simulink model "bicopter_startAngelo"  (R2026b)
settings: Solver=VariableStepAuto  StopTime=50
PreLoadFcn:
  | addpath("Support_Files/")
  | modelParams
model workspace (MAT data in the model file):
  TwinPivotDamping = 5.5e-05
  TwinThrustCoefficient = 0.9085
undefined symbols (not defined in the file or in its folder): battVoltage, MassVals, smiData, X, Y, Z
libraries: sm_lib x20, fl_lib x11, nesl_utility x4, sdl_lib x2, ee_lib x2, slpidlib x1, cstblocks_lti x1
(part 1 of 2)
settings Model: Creator=aredfear  LastModifiedBy=ayeo
settings RTWCC: GPUComputeCapability=5.0
settings SimscapeCC: SimscapeUseEnergyAccounting=off
settings ExplorerConfigSet: InternalSimMechanicsExplorerSettings=|
  | <ExplorerConfiguration>
  | 
  |   <canonicalview>default</canonicalview>
  | 
  |   <TilePanel>
  |     <TileInfo>
  |       <Tiles Columns="1" Count="1" Height="310" Rows="1" Width="757">
  |         <Row Weight="1"/>
  |         <Column Weight="1"/>
  |         <Tile Height="1" Width="1" X="0" Y="0"/>
  |       </Tiles>
  |     </TileInfo>
  |     <SceneInfo>
  |       <SceneViewer>
  |         <IsThisViewStd>
  |           <IsStandardView>off</IsStandardView>
  |           <StandardViewName>Front</StandardViewName>
  |         </IsThisViewStd>
  |         <BGColor>
  |           <R>1</R>
  |           <G>1</G>
  |           <B>1</B>
  |           <A>1</A>
  |         </BGColor>
  |         <Camera>
  |           <DoPerspective>off</DoPerspective>
  |           <Position>
  |             <X>0.27879065959295879</X>
  |             <Y>-2.0709674160574254</Y>
  |             <Z>0.54548044125818385</Z>
  |           </Position>
  |           <Center>
  |             <X>-0.0098286292275114144</X>
  |             <Y>0.00045902017735405254</Y>
  |             <Z>0.055789039094021275</Z>
  |           </Center>
  |           <Up>
  |             <X>-0.012086790678740725</X>
  |             <Y>0.22844965094818886</Y>
  |             <Z>0.97348069650750602</Z>
  |           </Up>
  |           <XLim>0.10544914134742404</XLim>
  |           <YLim>0.10544914134742404</YLim>
  |           <ViewLimDist>0.01</ViewLimDist>
  |         </Camera>
  |       </SceneViewer>
  |     </SceneInfo>
  |   </TilePanel>
  | 
  |   <MechEditorPanel>
  |     <GfxPanelCameraMap/>
  |     <Cameras/>
  |     <VideoCreator>
  |       <IncludeTiles>All</IncludeTiles>
  |       <IncludeTime>on</IncludeTime>
  |       <IncludeWorldFrame>off</IncludeWorldFrame>
  |       <PlaybackSpeedRatio>1</PlaybackSpeedRatio>
  |       <FrameRate>30</FrameRate>
  |       <FrameSize>auto</FrameSize>
  |       <VideoFormat>UncompressedAVI</VideoFormat>
  |     </VideoCreator>
  |   </MechEditorPanel>
  | 
  |   <PlaybackSettings>
  |     <PlaybackSpeedFactor>1</PlaybackSpeedFactor>
  |   </PlaybackSettings>
  | 
  | </ExplorerConfiguration>

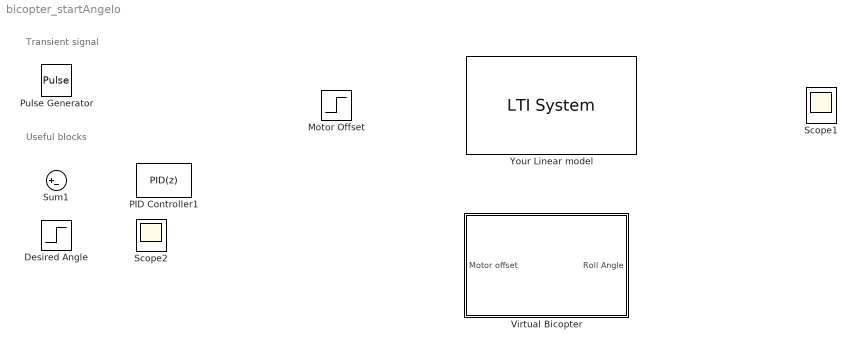
== system bicopter_startAngelo ==
  note: Useful blocks
  note: Transient signal
  Desired Angle : Step  FinalValue=20 * pi / 180  SampleTime=0
  Motor Offset : Step  FinalValue=5  SampleTime=0
  PID Controller1 : slpidlib/PID Controller  Controller=PID  Form=Parallel  TimeDomain=Discrete-time  UseExternalTs=off  SampleTime=0.001  IntegratorMethod=Forward Euler  FilterMethod=Forward Euler  ControllerParametersSource=internal  P=1  I=1  UseKiTs=off  D=0  UseExternalDerivativeSource=off  N=100  UseFilter=on  TunerSelectOption=Transfer Function Based (PID Tuner App)  InitialConditionSource=internal  InitialConditionForIntegrator=0  InitialConditionForFilter=0  DifferentiatorICPrevScaledInput=0  ExternalReset=none  TrackingMode=off  Kt=1  LimitOutput=on  SatLimitsSource=internal  UpperSaturationLimit=30  LowerSaturationLimit=-30  LinearizeAsGain=on  AntiWindupMode=clamping  Kb=1  LimitIntegrator=off  UpperIntegratorSaturationLimit=inf  LowerIntegratorSaturationLimit=-inf  POutMin=[]  POutMax=[]  IOutMin=[]  IOutMax=[]  DOutMin=[]  DOutMax=[]  NOutMin=[]  NOutMax=[]  SumOutMin=[]  SumOutMax=[]  SaturationOutMin=[]  SaturationOutMax=[]  PParamMin=[]  PParamMax=[]  IParamMin=[]  IParamMax=[]  DParamMin=[]  DParamMax=[]  NParamMin=[]  NParamMax=[]  KbParamMin=[]  KbParamMax=[]  KtParamMin=[]  KtParamMax=[]  KbOutMin=[]  KbOutMax=[]  KtOutMin=[]  KtOutMax=[]  IntegratorOutMin=[]  IntegratorOutMax=[]  FilterOutMin=[]  FilterOutMax=[]  SumI1OutMin=[]  SumI1OutMax=[]  SumI2OutMin=[]  SumI2OutMax=[]  SumI3OutMin=[]  SumI3OutMax=[]  SumI4OutMin=[]  SumI4OutMax=[]  SumDOutMin=[]  SumDOutMax=[]  DifferentiatorOutMin=[]  DifferentiatorOutMax=[]  FilterDiffOutCoefMin=[]  FilterDiffOutCoefMax=[]  ReciprocalOutMin=[]  ReciprocalOutMax=[]  SumDenOutMin=[]  SumDenOutMax=[]  SumNumOutMin=[]  SumNumOutMax=[]  DivideOutMin=[]  DivideOutMax=[]  UdiffTsProdOutMin=[]  UdiffTsProdOutMax=[]  NTsProdOutMin=[]  NTsProdOutMax=[]  UintegralTsProdOutMin=[]  UintegralTsProdOutMax=[]  UngainTsProdOutMin=[]  UngainTsProdOutMax=[]  ClampingZeroOutDataTypeStr=Inherit: Inherit via back propagation  ClampingZeroOutMin=[]  ClampingZeroOutMax=[]  FilterDenConstantOutDataTypeStr=Inherit: Inherit via back propagation  FilterDenConstantOutMin=[]  FilterDenConstantOutMax=[]  PCopyOutDataTypeStr=Inherit: Inherit via back propagation  PCopyOutMin=[]  PCopyOutMax=[]  NCopyOutDataTypeStr=Inherit: Inherit via back propagation  NCopyOutMin=[]  NCopyOutMax=[]  IntegratorContinuousStateAttributes=''  IntegratorStateMustResolveToSignalObject=off  IntegratorRTWStateStorageClass=Auto  FilterContinuousStateAttributes=''  FilterStateMustResolveToSignalObject=off  FilterRTWStateStorageClass=Auto  ParallelPVariant=InternalParameters  IdealPVariant=Disabled  IVariant=InternalParameters  DVariant=InternalParameters  IntegratorVariant=Discrete  SatVariant=Enabled  AWVariant=DiscClampingParallel  PCopyVariant=Disabled  TRVariant=Disabled  FdbkBlocksVariant=Forward  IdealPFdbkVariant=Disabled  SatFdbkVariant=Disabled  DerivativeFilterVariant=ForwardEulerFilter  NVariant=InternalParameters  NCopyVariant=Disabled  FilterICVariant=InternalICsFilter  IntegratorICVariant=InternalICs  ExternalResetVariant=Disabled  TRSumVariant=Passthrough  SumFdbkVariant=Disabled  SumVariant=Sum_PID  TsampFilterVariant=InternalTs  TsampNgainVariant=Passthrough  TsampIntegralVariant=Disabled_SignalSpec  ExternalSaturationOutDataTypeStr=Inherit: Same as second input  DerivativeSourceVariant=ErrorSignal  PreIntVariant=InternalPreInt
  Pulse Generator : DiscretePulseGenerator  PulseType=Time based  Amplitude=20 * pi / 180  Period=50  PulseWidth=50  PhaseDelay=10
  Scope1 : Scope
      settings: ActiveDisplayYMinimum=-0.043692144868254922  ActiveDisplayYMaximum=0.39270562765076822
  Scope2 : Scope
      settings: DataLoggingVariableName=ScopeData2
  Sum1 : Sum  Inputs=|+-
  Virtual Bicopter : Subsystem
      mask Display: image('bicopter.png');
  Your Linear model : cstblocks_lti/LTI System  sys=myModel  IC=[]  PadeOrder=0

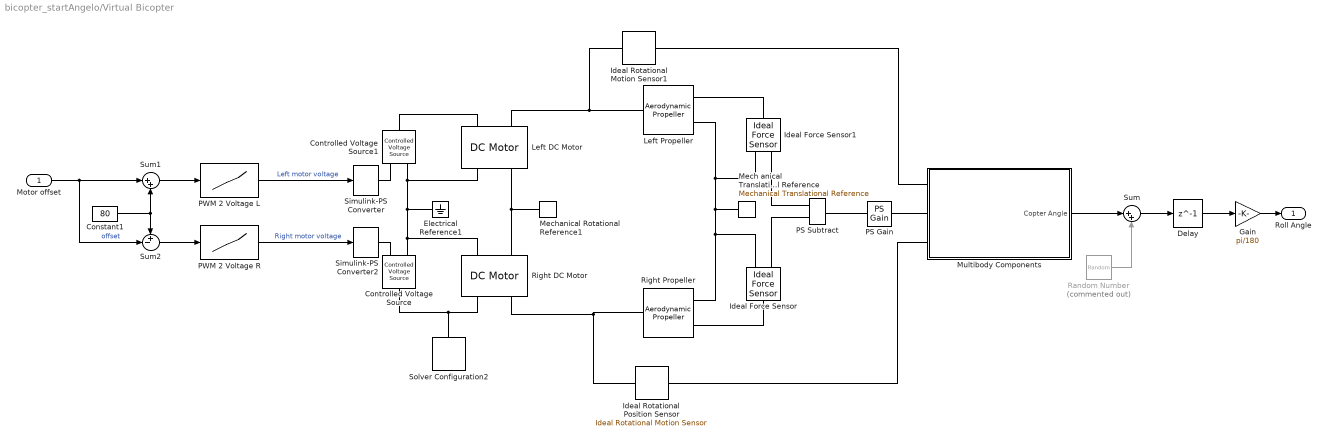
== system bicopter_startAngelo/Virtual Bicopter ==
  Motor offset : Inport
  Constant1 : Constant  Value=80
  Controlled Voltage Source : fl_lib/Electrical/Electrical Sources/Controlled Voltage Source
  Controlled Voltage Source1 : fl_lib/Electrical/Electrical Sources/Controlled Voltage Source
  Delay : Delay  DelayLength=1
  Electrical Reference1 : fl_lib/Electrical/Electrical Elements/Electrical Reference
  Gain : Gain  Gain=pi/180
  Ideal Force Sensor : fl_lib/Mechanical/Mechanical Sensors/Ideal Force Sensor
  Ideal Force Sensor1 : fl_lib/Mechanical/Mechanical Sensors/Ideal Force Sensor
  Ideal Rotational Motion Sensor1 : fl_lib/Mechanical/Mechanical Sensors/Ideal Rotational Motion Sensor  reference=foundation.enum.MeasurementReference.absolute  acceleration_port=false  velocity_port=false  position_port=true  wrap_angle=simscape.enum.onoff.off  offset=0 rad
  Ideal Rotational Position Sensor : fl_lib/Mechanical/Mechanical Sensors/Ideal Rotational Motion Sensor  reference=foundation.enum.MeasurementReference.absolute  acceleration_port=false  velocity_port=false  position_port=true  wrap_angle=false  offset=0 rad
  Left Propeller : sdl_lib/Engines & Motors/Aerodynamic Propeller  parameterization=sdl.enum.AerodynamicPropellerParameterization.Constant  enable_collective_pitch_control=false  enable_transverse_flow=false  direction=sdl.enum.PropellerDirection.Positive  root_pitch=0 deg  D=.02 m  kt_const=TwinThrustCoefficient  kp_const=0.13  kt_poly_fixed=[.002, .0006, -.0509, .0617]  kp_poly_fixed=[-.0752, .0577, -.0622, .16]  pitch_angle_TLU=[-15, 15, 25, 35, 45] deg  kt_poly_TLU=[.0002, -.00041, -.036, .03; .00026, -.00056, -.048, .04; .002, .00063, -.051, .062; .0014, -.0016, -.048, .087; .00087, -.0036, -.041, .12]  kp_poly_TLU=[-.1, .031, .0055, .088; -.081, -.025, .0044, .07; -.075, .058, -.062, .16; -.052, .065, -.08, .3; -.031, .057, -.069, .4]  J_TLU=[.01, .3, .625, 1.55, 2, 2.6]  kt_TLU_1D=[.0614, .0473, .0318, -.0127, -.0343, -.063]  kp_TLU_1D=[.1496, .1314, .116, -.0521, -.1503, -.2813]  kt_TLU_2D=[.00019, .013, .0048, -.017, -.03, -.045; .00039, .025, .0096, -.037, -.06, -.09; .00061, .047, .032, -.013, -.034, -.063; .00086, .072, .057, .014, -.0076, -.036; .12, .104, .09, .049, .029, .0019]  kp_TLU_2D=[.029, .029, .016, .06, .009, -.16; .059, .054, .031, -.12, -.19, -.29; .15, .13, .12, -.052, -.15, -.28; .26, .24, .22, .097, -.04, -.25; .39, .39, .38, .32, .24, .062]  beta_TLU=linspace(0, 360, 10) deg  Ct_TLU_1D=0.035 * sind(linspace(0, 360, 10) - 200)  Cq_TLU_1D=0.010 * sind(linspace(0, 360, 10) - 200)  Ct_TLU_2D=[0.01 * sind(linspace(0, 360, 10) - 200); 0.020 * sind(linspace(0, 360, 10) - 200); 0.035 * sind(linspace(0, 360, 10) - 200); 0.04 * sind(linspace(0, 360, 10) - 200); 0.06 * sind(linspace(0, 360, 10) - 200)]  Cq_TLU_2D=[0.0005 * sind(linspace(0, 360, 10) - 200); 0.0015 * sind(linspace(0, 360, 10) - 200); 0.0025 * sind(linspace(0, 360, 10) - 200); 0.0035 * sind(linspace(0, 360, 10) - 200); 0.0045 * sind(linspace(0, 360, 10) - 200)]  n_blades=2  radial_TLU=[.1, .12, .2, .4, .6, .8, 1]  twist_TLU=[30, 35, 50, 30, 20, 15, 10] deg  chord_TLU=[.0676, .0666, .0824, .1025, .0885, .0598, .0133]  alpha_TLU=-180 : 10 : 180 deg  Cl_TLU=[.1326, .1326, .1274, .1274, .1274, .1274, .1274; .3626, .3626, .5002, .5002, .5002, .5002, .5002; .5528, .5528, .8007, .8007, .8007, .8007, .8007; .7256, .7256, 1.0125, 1.0125, 1.0125, 1.0125, 1.0125; .8016, .8016, 1.1556, 1.1556, 1.1556, 1.1556, 1.1556; .7873, .7873, 1.1604, 1.1604, 1.1604, 1.1604, 1.1604; .7031, .7031, 1.0493, 1.0493, 1.0493, 1.0493, 1.0493; .5423, .5423, .7973, .7973, .7973, .7973, .7973; .3537, .3537, .4332, .4332, .4332, .4332, .4332; .1155, .1155, -.0376, -.0376, -.0376, -.0376, -.0376; -.1045, -.1045, -.4096, -.4096, -.4096, -.4096, -.4096; -.2999, -.2999, -.672, -.672, -.672, -.672, -.672; -.4401, -.4401, -.9343, -.9343, -.9343, -.9343, -.9343; -.5186, -.5186, -1.0477, -1.0477, -1.0477, -1.0477, -1.0477; -.5303, -.5303, -1.0387, -1.0387, -1.0387, -1.0387, -1.0387; -.5073, -.5073, -.9565, -.9565, -.9565, -.9565, -.9565; -.442, -.442, -.7713, -.7713, -.7713, -.7713, -.7713; -.2658, -.2658, -.4832, -.4832, -.4832, -.4832, -.4832; .4109, .4109, .3629, .3629, .3629, .3629, .3629; 1.1635, 1.1635, 1.3779, 1.3779, 1.3779, 1.3779, 1.3779; 1.2412, 1.2412, 1.4033, 1.4033, 1.4033, 1.4033, 1.4033; .7434, .7434, 1.3453, 1.3453, 1.3453, 1.3453, 1.3453; .7908, .7908, 1.2862, 1.2862, 1.2862, 1.2862, 1.2862; .7525, .7525, 1.1562, 1.1562, 1.1562, 1.1562, 1.1562; .6722, .6722, .9487, .9487, .9487, .9487, .9487; .5324, .5324, .7047, .7047, .7047, .7047, .7047; .3365, .3365, .382, .382, .382, .382, .382; .0529, .0529, -.0229, -.0229, -.0229, -.0229, -.0229; -.2728, -.2728, -.316, -.316, -.316, -.316, -.316; -.4135, -.4135, -.6195, -.6195, -.6195, -.6195, -.6195; -.5087, -.5087, -.7847, -.7847, -.7847, -.7847, -.7847; -.5342, -.5342, -.8419, -.8419, -.8419, -.8419, -.8419; -.5166, -.5166, -.7658, -.7658, -.7658, -.7658, -.7658; -.4321, -.4321, -.5707, -.5707, -.5707, -.5707, -.5707; -.2864, -.2864, -.3098, -.3098, -.3098, -.3098, -.3098; -.1073, -.1073, -.0893, -.0893, -.0893, -.0893, -.0893; .1326, .1326, .1274, .1274, .1274, .1274, .1274]  Cd_TLU=[.0055, .0055, .3904, .3904, .3904, .3904, .3904; .0774, .0774, .449, .449, .449, .449, .449; .2412, .2412, .5915, .5915, .5915, .5915, .5915; .4342, .4342, .8307, .8307, .8307, .8307, .8307; .679, .679, 1.0909, 1.0909, 1.0909, 1.0909, 1.0909; .9003, .9003, 1.3868, 1.3868, 1.3868, 1.3868, 1.3868; 1.0825, 1.0825, 1.6565, 1.6565, 1.6565, 1.6565, 1.6565; 1.2281, 1.2281, 1.875, 1.875, 1.875, 1.875, 1.875; 1.3205, 1.3205, 2.017, 2.017, 2.017, 2.017, 2.017; 1.3234, 1.3234, 2.0407, 2.0407, 2.0407, 2.0407, 2.0407; 1.2391, 1.2391, 1.9513, 1.9513, 1.9513, 1.9513, 1.9513; 1.0963, 1.0963, 1.7643, 1.7643, 1.7643, 1.7643, 1.7643; .8978, .8978, 1.5048, 1.5048, 1.5048, 1.5048, 1.5048; .6525, .6525, 1.2281, 1.2281, 1.2281, 1.2281, 1.2281; .4203, .4203, .838, .838, .838, .838, .838; .2428, .2428, .5434, .5434, .5434, .5434, .5434; .0951, .0951, .2517, .2517, .2517, .2517, .2517; .0292, .0292, .0698, .0698, .0698, .0698, .0698; .0148, .0148, .0267, .0267, .0267, .0267, .0267; .0808, .0808, .0509, .0509, .0509, .0509, .0509; .2429, .2429, .1561, .1561, .1561, .1561, .1561; .5019, .5019, .3927, .3927, .3927, .3927, .3927; .7217, .7217, .7438, .7438, .7438, .7438, .7438; .9336, .9336, 1.1277, 1.1277, 1.1277, 1.1277, 1.1277; 1.0984, 1.0984, 1.4838, 1.4838, 1.4838, 1.4838, 1.4838; 1.2274, 1.2274, 1.7877, 1.7877, 1.7877, 1.7877, 1.7877; 1.3016, 1.3016, 1.9779, 1.9779, 1.9779, 1.9779, 1.9779; 1.3305, 1.3305, 2.0516, 2.0516, 2.0516, 2.0516, 2.0516; 1.2889, 1.2889, 1.9974, 1.9974, 1.9974, 1.9974, 1.9974; 1.1677, 1.1677, 1.8463, 1.8463, 1.8463, 1.8463, 1.8463; 1.0076, 1.0076, 1.5699, 1.5699, 1.5699, 1.5699, 1.5699; .8068, .8068, 1.2596, 1.2596, 1.2596, 1.2596, 1.2596; .5688, .5688, .9493, .9493, .9493, .9493, .9493; .3604, .3604, .6154, .6154, .6154, .6154, .6154; .1802, .1802, .5015, .5015, .5015, .5015, .5015; .0699, .0699, .4265, .4265, .4265, .4265, .4265; .0055, .0055, .3904, .3904, .3904, .3904, .3904]  interp_method=simscape.enum.interpolation.linear  extrap_method=simscape.enum.extrapolation.linear  n_blade_discretization=20  n_azimuthal_discretization=10  density_spec=foundation.enum.constant_variable.constant  rho=1.225 kg/m^3  rotational_ports=sdl.enum.ConnectionType.Conserving  translational_ports=sdl.enum.ConnectionType.Conserving  model_inertia=false  propeller_inertia=1e-6 kg*m^2  propeller_mass=1e-4 kg  efficiency_sensor=false  n_thr=0.001 Hz  k_thr=0.001  P_thr=0.01 W  operation_check=simscape.enum.assert.action.warn  expose_port_C=false  w_specify=off  w_priority=None  w=0 rad/s  w_nominal_specify=on  w_nominal_value=1  w_nominal_unit=rad/s  Q_specify=off  Q_priority=None  Q=0 N*m  Q_nominal_specify=off  Q_nominal_value=1  Q_nominal_unit=N*m  v_specify=off  v_priority=None  v=0 m/s  v_nominal_specify=off  v_nominal_value=1  v_nominal_unit=m/s  thrust_specify=off  thrust_priority=None  thrust=0 N  thrust_nominal_specify=on  thrust_nominal_value=1  thrust_nominal_unit=N
  Left DC Motor : ee_lib/Electromechanical/Brushed Motors/DC Motor  field_option=ee.enum.field_option.pm  Rf=100 Ohm  Lf=1 H  Laf=0.15 H  If0=0 A  parameterization=ee.enum.dcparam_option.circuit_param  Ra=1.9 Ohm  La=12e-6 H  emf_or_torque=ee.enum.emf_or_torque.kv  Kv=0.072e-3 V/rpm  Ki=6.876e-4 N*m/A  T_stall=0.24e-3 N*m  w_max=19100 rpm  w_rated=15000 rpm  P_rated=0.08 W  V_rated=1.5 V  lam_param=ee.enum.lam_param.damping  i_noload=0 A  V_i_noload=1.5 V  J=0.01 cm^2*g  lam=0 N*m*s/rad  speed0=0 rpm  alpha=3.93e-3 1/K  Tmeas=25 degC  thermal_mass=100 J/K  initial_temperature=25 degC
  Mech anical Translational Reference : fl_lib/Mechanical/Translational Elements/Mechanical Translational Reference
  Mechanical Rotational Reference1 : fl_lib/Mechanical/Rotational Elements/Mechanical Rotational Reference
  Multibody Components : Subsystem
  PS Gain : fl_lib/Physical Signals/Functions/PS Gain  gain=10 cm
  PS Subtract : fl_lib/Physical Signals/Functions/PS Subtract
  PWM 2 Voltage L : Lookup_n-D  NumberOfTableDimensions=1  BreakpointsForDimension1=[0, 255]  Table=[0, battVoltage]  ExtrapMethod=Clip  InternalRulePriority=Speed  RndMeth=Simplest
  PWM 2 Voltage R : Lookup_n-D  NumberOfTableDimensions=1  BreakpointsForDimension1=[0, 255]  Table=[0, battVoltage]  ExtrapMethod=Clip  InternalRulePriority=Speed  RndMeth=Simplest
  Random Number : RandomNumber  Commented=on  Variance=0.1
  Right Propeller : sdl_lib/Engines & Motors/Aerodynamic Propeller  parameterization=sdl.enum.AerodynamicPropellerParameterization.Constant  enable_collective_pitch_control=false  enable_transverse_flow=false  direction=sdl.enum.PropellerDirection.Positive  root_pitch=0 deg  D=.02 m  kt_const=TwinThrustCoefficient  kp_const=0.13  kt_poly_fixed=[.002, .0006, -.0509, .0617]  kp_poly_fixed=[-.0752, .0577, -.0622, .16]  pitch_angle_TLU=[-15, 15, 25, 35, 45] deg  kt_poly_TLU=[.0002, -.00041, -.036, .03; .00026, -.00056, -.048, .04; .002, .00063, -.051, .062; .0014, -.0016, -.048, .087; .00087, -.0036, -.041, .12]  kp_poly_TLU=[-.1, .031, .0055, .088; -.081, -.025, .0044, .07; -.075, .058, -.062, .16; -.052, .065, -.08, .3; -.031, .057, -.069, .4]  J_TLU=[.01, .3, .625, 1.55, 2, 2.6]  kt_TLU_1D=[.0614, .0473, .0318, -.0127, -.0343, -.063]  kp_TLU_1D=[.1496, .1314, .116, -.0521, -.1503, -.2813]  kt_TLU_2D=[.00019, .013, .0048, -.017, -.03, -.045; .00039, .025, .0096, -.037, -.06, -.09; .00061, .047, .032, -.013, -.034, -.063; .00086, .072, .057, .014, -.0076, -.036; .12, .104, .09, .049, .029, .0019]  kp_TLU_2D=[.029, .029, .016, .06, .009, -.16; .059, .054, .031, -.12, -.19, -.29; .15, .13, .12, -.052, -.15, -.28; .26, .24, .22, .097, -.04, -.25; .39, .39, .38, .32, .24, .062]  beta_TLU=linspace(0, 360, 10) deg  Ct_TLU_1D=0.035 * sind(linspace(0, 360, 10) - 200)  Cq_TLU_1D=0.010 * sind(linspace(0, 360, 10) - 200)  Ct_TLU_2D=[0.01 * sind(linspace(0, 360, 10) - 200); 0.020 * sind(linspace(0, 360, 10) - 200); 0.035 * sind(linspace(0, 360, 10) - 200); 0.04 * sind(linspace(0, 360, 10) - 200); 0.06 * sind(linspace(0, 360, 10) - 200)]  Cq_TLU_2D=[0.0005 * sind(linspace(0, 360, 10) - 200); 0.0015 * sind(linspace(0, 360, 10) - 200); 0.0025 * sind(linspace(0, 360, 10) - 200); 0.0035 * sind(linspace(0, 360, 10) - 200); 0.0045 * sind(linspace(0, 360, 10) - 200)]  n_blades=2  radial_TLU=[.1, .12, .2, .4, .6, .8, 1]  twist_TLU=[30, 35, 50, 30, 20, 15, 10] deg  chord_TLU=[.0676, .0666, .0824, .1025, .0885, .0598, .0133]  alpha_TLU=-180 : 10 : 180 deg  Cl_TLU=[.1326, .1326, .1274, .1274, .1274, .1274, .1274; .3626, .3626, .5002, .5002, .5002, .5002, .5002; .5528, .5528, .8007, .8007, .8007, .8007, .8007; .7256, .7256, 1.0125, 1.0125, 1.0125, 1.0125, 1.0125; .8016, .8016, 1.1556, 1.1556, 1.1556, 1.1556, 1.1556; .7873, .7873, 1.1604, 1.1604, 1.1604, 1.1604, 1.1604; .7031, .7031, 1.0493, 1.0493, 1.0493, 1.0493, 1.0493; .5423, .5423, .7973, .7973, .7973, .7973, .7973; .3537, .3537, .4332, .4332, .4332, .4332, .4332; .1155, .1155, -.0376, -.0376, -.0376, -.0376, -.0376; -.1045, -.1045, -.4096, -.4096, -.4096, -.4096, -.4096; -.2999, -.2999, -.672, -.672, -.672, -.672, -.672; -.4401, -.4401, -.9343, -.9343, -.9343, -.9343, -.9343; -.5186, -.5186, -1.0477, -1.0477, -1.0477, -1.0477, -1.0477; -.5303, -.5303, -1.0387, -1.0387, -1.0387, -1.0387, -1.0387; -.5073, -.5073, -.9565, -.9565, -.9565, -.9565, -.9565; -.442, -.442, -.7713, -.7713, -.7713, -.7713, -.7713; -.2658, -.2658, -.4832, -.4832, -.4832, -.4832, -.4832; .4109, .4109, .3629, .3629, .3629, .3629, .3629; 1.1635, 1.1635, 1.3779, 1.3779, 1.3779, 1.3779, 1.3779; 1.2412, 1.2412, 1.4033, 1.4033, 1.4033, 1.4033, 1.4033; .7434, .7434, 1.3453, 1.3453, 1.3453, 1.3453, 1.3453; .7908, .7908, 1.2862, 1.2862, 1.2862, 1.2862, 1.2862; .7525, .7525, 1.1562, 1.1562, 1.1562, 1.1562, 1.1562; .6722, .6722, .9487, .9487, .9487, .9487, .9487; .5324, .5324, .7047, .7047, .7047, .7047, .7047; .3365, .3365, .382, .382, .382, .382, .382; .0529, .0529, -.0229, -.0229, -.0229, -.0229, -.0229; -.2728, -.2728, -.316, -.316, -.316, -.316, -.316; -.4135, -.4135, -.6195, -.6195, -.6195, -.6195, -.6195; -.5087, -.5087, -.7847, -.7847, -.7847, -.7847, -.7847; -.5342, -.5342, -.8419, -.8419, -.8419, -.8419, -.8419; -.5166, -.5166, -.7658, -.7658, -.7658, -.7658, -.7658; -.4321, -.4321, -.5707, -.5707, -.5707, -.5707, -.5707; -.2864, -.2864, -.3098, -.3098, -.3098, -.3098, -.3098; -.1073, -.1073, -.0893, -.0893, -.0893, -.0893, -.0893; .1326, .1326, .1274, .1274, .1274, .1274, .1274]  Cd_TLU=[.0055, .0055, .3904, .3904, .3904, .3904, .3904; .0774, .0774, .449, .449, .449, .449, .449; .2412, .2412, .5915, .5915, .5915, .5915, .5915; .4342, .4342, .8307, .8307, .8307, .8307, .8307; .679, .679, 1.0909, 1.0909, 1.0909, 1.0909, 1.0909; .9003, .9003, 1.3868, 1.3868, 1.3868, 1.3868, 1.3868; 1.0825, 1.0825, 1.6565, 1.6565, 1.6565, 1.6565, 1.6565; 1.2281, 1.2281, 1.875, 1.875, 1.875, 1.875, 1.875; 1.3205, 1.3205, 2.017, 2.017, 2.017, 2.017, 2.017; 1.3234, 1.3234, 2.0407, 2.0407, 2.0407, 2.0407, 2.0407; 1.2391, 1.2391, 1.9513, 1.9513, 1.9513, 1.9513, 1.9513; 1.0963, 1.0963, 1.7643, 1.7643, 1.7643, 1.7643, 1.7643; .8978, .8978, 1.5048, 1.5048, 1.5048, 1.5048, 1.5048; .6525, .6525, 1.2281, 1.2281, 1.2281, 1.2281, 1.2281; .4203, .4203, .838, .838, .838, .838, .838; .2428, .2428, .5434, .5434, .5434, .5434, .5434; .0951, .0951, .2517, .2517, .2517, .2517, .2517; .0292, .0292, .0698, .0698, .0698, .0698, .0698; .0148, .0148, .0267, .0267, .0267, .0267, .0267; .0808, .0808, .0509, .0509, .0509, .0509, .0509; .2429, .2429, .1561, .1561, .1561, .1561, .1561; .5019, .5019, .3927, .3927, .3927, .3927, .3927; .7217, .7217, .7438, .7438, .7438, .7438, .7438; .9336, .9336, 1.1277, 1.1277, 1.1277, 1.1277, 1.1277; 1.0984, 1.0984, 1.4838, 1.4838, 1.4838, 1.4838, 1.4838; 1.2274, 1.2274, 1.7877, 1.7877, 1.7877, 1.7877, 1.7877; 1.3016, 1.3016, 1.9779, 1.9779, 1.9779, 1.9779, 1.9779; 1.3305, 1.3305, 2.0516, 2.0516, 2.0516, 2.0516, 2.0516; 1.2889, 1.2889, 1.9974, 1.9974, 1.9974, 1.9974, 1.9974; 1.1677, 1.1677, 1.8463, 1.8463, 1.8463, 1.8463, 1.8463; 1.0076, 1.0076, 1.5699, 1.5699, 1.5699, 1.5699, 1.5699; .8068, .8068, 1.2596, 1.2596, 1.2596, 1.2596, 1.2596; .5688, .5688, .9493, .9493, .9493, .9493, .9493; .3604, .3604, .6154, .6154, .6154, .6154, .6154; .1802, .1802, .5015, .5015, .5015, .5015, .5015; .0699, .0699, .4265, .4265, .4265, .4265, .4265; .0055, .0055, .3904, .3904, .3904, .3904, .3904]  interp_method=simscape.enum.interpolation.linear  extrap_method=simscape.enum.extrapolation.linear  n_blade_discretization=20  n_azimuthal_discretization=10  density_spec=foundation.enum.constant_variable.constant  rho=1.225 kg/m^3  rotational_ports=sdl.enum.ConnectionType.Conserving  translational_ports=sdl.enum.ConnectionType.Conserving  model_inertia=false  propeller_inertia=1e-6 kg*m^2  propeller_mass=1e-4 kg  efficiency_sensor=false  n_thr=0.001 Hz  k_thr=0.001  P_thr=0.01 W  operation_check=simscape.enum.assert.action.warn  expose_port_C=false  w_specify=off  w_priority=None  w=0 rad/s  w_nominal_specify=on  w_nominal_value=1  w_nominal_unit=rad/s  Q_specify=off  Q_priority=None  Q=0 N*m  Q_nominal_specify=off  Q_nominal_value=1  Q_nominal_unit=N*m  v_specify=off  v_priority=None  v=0 m/s  v_nominal_specify=off  v_nominal_value=1  v_nominal_unit=m/s  thrust_specify=off  thrust_priority=None  thrust=0 N  thrust_nominal_specify=on  thrust_nominal_value=1  thrust_nominal_unit=N
  Right DC Motor : ee_lib/Electromechanical/Brushed Motors/DC Motor  field_option=ee.enum.field_option.pm  Rf=100 Ohm  Lf=1 H  Laf=0.15 H  If0=0 A  parameterization=ee.enum.dcparam_option.circuit_param  Ra=1.9 Ohm  La=12e-6 H  emf_or_torque=ee.enum.emf_or_torque.kv  Kv=0.072e-3 V/rpm  Ki=6.876e-4 N*m/A  T_stall=0.24e-3 N*m  w_max=19100 rpm  w_rated=15000 rpm  P_rated=0.08 W  V_rated=1.5 V  lam_param=ee.enum.lam_param.damping  i_noload=0 A  V_i_noload=1.5 V  J=0.01 cm^2*g  lam=0 N*m*s/rad  speed0=0 rpm  alpha=3.93e-3 1/K  Tmeas=25 degC  thermal_mass=100 J/K  initial_temperature=25 degC
  Simulink-PS Converter : nesl_utility/Simulink-PS Converter  PhysicalDomain=network_engine_domain  SubClassName=ps_input  LeftPortType=input  RightPortType=output  PseudoPeriodic=off  Frequencies=[]  NoiseDistribution=none  NoiseParameters=[]  Unit=1  AffineConversion=off  FilteringAndDerivatives=filter  SimscapeFilterOrder=2  InputFilterTimeConstant=0.001  UdotUserProvided=1
  Simulink-PS Converter2 : nesl_utility/Simulink-PS Converter  PhysicalDomain=network_engine_domain  SubClassName=ps_input  LeftPortType=input  RightPortType=output  PseudoPeriodic=off  Frequencies=[]  NoiseDistribution=none  NoiseParameters=[]  Unit=1  AffineConversion=off  FilteringAndDerivatives=filter  SimscapeFilterOrder=2  InputFilterTimeConstant=0.001  UdotUserProvided=1
  Solver Configuration2 : nesl_utility/Solver Configuration  PhysicalDomain=network_engine_domain  SubClassName=solver  LeftPortType=input  RightPortType=generic  Tones=[]  Harmonics=[]  SimulateNoise=off  Profile=off  UseLocalSampling=off  EnableSwitchedLinearOptims=on  FrequencyDomain=off  UseCCode=off  RelTol=0.001  AbsTol=0.001  MinStep=1e-09  ToWorkspace=off  RevertToSquareIcSolve=off  NumHomotopyIterations=100  PhasorMode=off  PhasorModeNumHarmonics=1  ConsistencySolver=NEWTON_XTOL_AFTER_FTOL  CanonicalOrdering=UNORDERED  OptimizeIntermediates=UNOPTIMIZED  MulticoreSolverChoice=BACKWARD_EULER  IndexReductionMethod=DerivativeReplacement  DoDC=off  ResidualTolerance=1e-09  ConsistencyTolSource=GLOBAL  ConsistencyAbsTol=0.001  ConsistencyRelTol=0.001  ConsistencyTolFactor=0.001  UseLocalSolver=off  LocalSolverChoice=NE_BACKWARD_EULER_ADVANCER  ResolveIndetEquations=on  FunctionEvalNumThread=1  LocalSolverSampleTime=0.001  DoFixedCost=off  MaxNonlinIter=3  MaxModeIter=2  ComputeImpulses=off  ImpulseIterations=2  LinearAlgebra=auto  LinearAlgebraNumThread=0  EquationFormulation=NE_TIME_EF  DelaysMemoryBudget=1024  AutomaticFiltering=on  FilteringTimeConstant=0.001  PartitionStorageMethod=AS_NEEDED  PartitionMemoryBudget=1024  PartitionMethod=BALANCED  MultibodyUseLocalSolver=off  MultibodyLocalSolverChoice=ODE1  MultibodyLocalSolverSampleTime=0.001
  Sum : Sum  Inputs=|++
  Sum1 : Sum  Inputs=|++
  Sum2 : Sum  Inputs=+-|
  Roll Angle : Outport
  wires:
  Motor offset/1 -> Sum1/1, Sum2/2  "offset"
  Sum2/1 -> PWM 2 Voltage R/1
  Sum1/1 -> PWM 2 Voltage L/1
  Constant1/1 -> Sum2/1, Sum1/2
  Random Number/1 -> Sum/2
  Sum/1 -> Delay/1
  Multibody Components/1(Copter Angle) -> Sum/1
  PWM 2 Voltage R/1 -> Simulink-PS Converter2/1  "Right motor voltage"
  PWM 2 Voltage L/1 -> Simulink-PS Converter/1  "Left motor voltage"
  Delay/1 -> Gain/1
  Gain/1 -> Roll Angle/1
  connections:
  Ideal Force Sensor/RConn1 -- Right Propeller/RConn2 -- Mech anical Translational Reference/LConn1 -- Ideal Force Sensor1/RConn1 -- Left Propeller/RConn2
  Controlled Voltage Source/RConn2 -- Right DC Motor/RConn1 -- Electrical Reference1/LConn1 -- Controlled Voltage Source1/RConn2 -- Left DC Motor/RConn1
  PS Subtract/RConn1 -- PS Gain/LConn1
  Right DC Motor/LConn2 -- Ideal Rotational Position Sensor/LConn1 -- Right Propeller/LConn1
  Simulink-PS Converter/RConn1 -- Controlled Voltage Source1/RConn1
  Controlled Voltage Source/LConn1 -- Solver Configuration2/RConn1 -- Right DC Motor/LConn1
  Right Propeller/RConn1 -- Ideal Force Sensor/LConn1
  Left Propeller/RConn1 -- Ideal Force Sensor1/LConn1
  Left DC Motor/LConn2 -- Ideal Rotational Motion Sensor1/LConn1 -- Left Propeller/LConn1
  Controlled Voltage Source1/LConn1 -- Left DC Motor/LConn1
  Controlled Voltage Source/RConn1 -- Simulink-PS Converter2/RConn1
  Mechanical Rotational Reference1/LConn1 -- Right DC Motor/RConn2 -- Left DC Motor/RConn2
  Ideal Rotational Motion Sensor1/RConn1 -- Multibody Components/LConn1
  PS Gain/RConn1 -- Multibody Components/LConn2
  PS Subtract/LConn1 -- Ideal Force Sensor1/RConn2
  PS Subtract/LConn2 -- Ideal Force Sensor/RConn2
  Multibody Components/LConn3 -- Ideal Rotational Position Sensor/RConn1

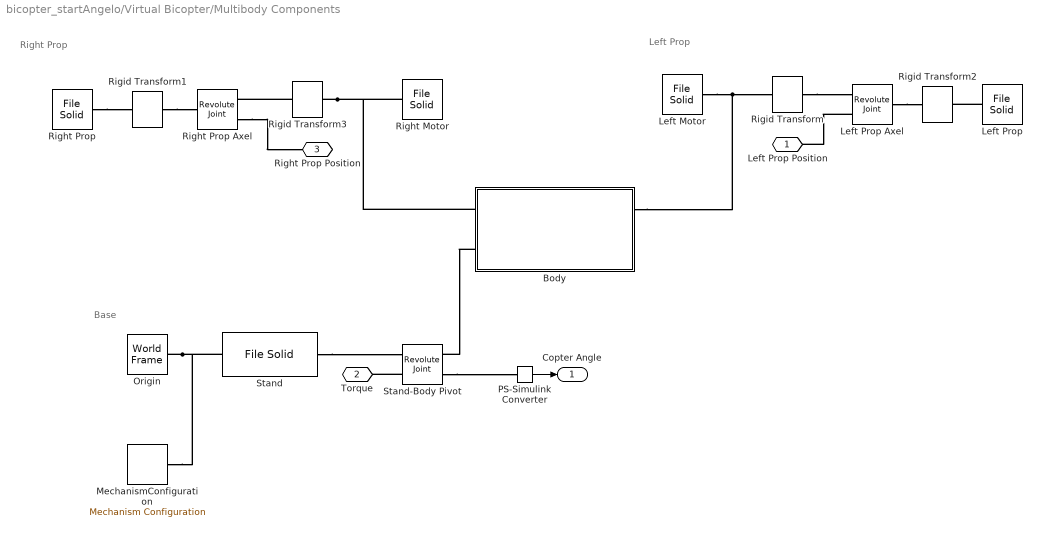
== system bicopter_startAngelo/Virtual Bicopter/Multibody Components ==
  note: Base
  note: Left Prop
  note: Right Prop
  Body : Subsystem
  Left Motor : sm_lib/Body Elements/File Solid  ExtGeomFileName=motor_Default_sldprt.STEP  UnitType=FromFile  ExtGeomFileUnits=m  StepReaderType=HEX  ExportConvexHullGeometry=off  InertiaType=CalculateFromGeometry  BasedOnType=Mass  Density=1000  DensityUnits=kg/m^3  Mass=MassVals.Motor  MassUnits=g  CenterOfMass=smiData.Solid(20).CoM  CenterOfMassUnits=mm  MomentsOfInertia=smiData.Solid(20).MoI  MomentsOfInertiaUnits=kg*mm^2  ProductsOfInertia=smiData.Solid(20).PoI  ProductsOfInertiaUnits=kg*mm^2  GraphicType=FromGeometry  MarkerShape=Sphere  MarkerSize=10  GraphicVisPropType=SimpleVisualProperties  GraphicDiffuseColor=[0.502 0.502 0.502]  GraphicOpacity=1  GraphicSpecularColor=[0.5 0.5 0.5 1.0]  GraphicAmbientColor=[0.15 0.15 0.15 1.0]  GraphicEmissiveColor=[0.0 0.0 0.0 1.0]  GraphicShininess=75  DoExposeReferenceFrame=off  SerializedFrames=|
      | <Frames>
      | 
      |   <Frame>
      |     <Id>Frame1</Id>
      |     <Value>
      |       <Name>Top</Name>
      |       <Origin>
      |         <Source>GeometricFeature</Source>
      |         <FeatureName>planar surface 1</FeatureName>
      |       </Origin>
      |       <PrimaryAxis>
      |         <DefinedDirection>+Y</DefinedDirection>
      |         <Source>ReferenceFrame</Source>
      |         <SourceDirection>+Z</SourceDirection>
      |         <FeatureName></FeatureName>
      |       </PrimaryAxis>
      |       <SecondaryAxis>
      |         <DefinedDirection>+X</DefinedDirection>
      |         <Source>ReferenceFrame</Source>
      |         <SourceDirection>-X</SourceDirection>
      |         <FeatureName></FeatureName>
      |       </SecondaryAxis>
      |     </Value>
      |   </Frame>
      | 
      | </Frames>
  Left Prop : sm_lib/Body Elements/File Solid  ExtGeomFileName=PropellerRED_Default_sldprt.STEP  UnitType=FromFile  ExtGeomFileUnits=m  StepReaderType=HEX  ExportConvexHullGeometry=off  InertiaType=CalculateFromGeometry  BasedOnType=Mass  Density=1000  DensityUnits=kg/m^3  Mass=MassVals.Prop  MassUnits=g  CenterOfMass=smiData.Solid(2).CoM  CenterOfMassUnits=mm  MomentsOfInertia=smiData.Solid(2).MoI  MomentsOfInertiaUnits=kg*mm^2  ProductsOfInertia=smiData.Solid(2).PoI  ProductsOfInertiaUnits=kg*mm^2  GraphicType=FromGeometry  MarkerShape=Sphere  MarkerSize=10  GraphicVisPropType=SimpleVisualProperties  GraphicDiffuseColor=[1 0 0]  GraphicOpacity=1  GraphicSpecularColor=[0.5 0.5 0.5 1.0]  GraphicAmbientColor=[0.15 0.15 0.15 1.0]  GraphicEmissiveColor=[0.0 0.0 0.0 1.0]  GraphicShininess=75  DoExposeReferenceFrame=off  SerializedFrames=|
      | <Frames>
      | 
      |   <Frame>
      |     <Id>Frame1</Id>
      |     <Value>
      |       <Name>Base</Name>
      |       <Origin>
      |         <Source>GeometricFeature</Source>
      |         <FeatureName>planar surface 3</FeatureName>
      |       </Origin>
      |       <PrimaryAxis>
      |         <DefinedDirection>+Z</DefinedDirection>
      |         <Source>ReferenceFrame</Source>
      |         <SourceDirection>+Z</SourceDirection>
      |         <FeatureName></FeatureName>
      |       </PrimaryAxis>
      |       <SecondaryAxis>
      |         <DefinedDirection>+X</DefinedDirection>
      |         <Source>ReferenceFrame</Source>
      |         <SourceDirection>+X</SourceDirection>
      |         <FeatureName></FeatureName>
      |       </SecondaryAxis>
      |     </Value>
      |   </Frame>
      | 
      | </Frames>
  Left Prop Axel : sm_lib/Joints/Revolute Joint  JointMode=Normal  CompositeWrenchDir=FollowerOnBase  CompositeWrenchFrame=BaseFrame  SenseConstraintForce=off  SenseConstraintTorque=off  SenseTotalForce=off  SenseTotalTorque=off  PositionTargetSpecify=on  PositionTargetPriority=Low  PositionTargetValue=0  PositionTargetValueUnits=deg  VelocityTargetSpecify=off  VelocityTargetPriority=High  VelocityTargetValue=0  VelocityTargetValueUnits=deg/s  EquilibriumPosition=0  EquilibriumPositionUnits=deg  SpringStiffness=0  SpringStiffnessUnits=N*m/deg  DampingCoefficient=0  DampingCoefficientUnits=N*m/(deg/s)  LowerLimitSpecify=off  LowerLimitBound=-90  LowerLimitBoundUnits=deg  LowerLimitStiffness=1e4  LowerLimitStiffnessUnits=N*m/deg  LowerLimitDamping=10  LowerLimitDampingUnits=N*m/(deg/s)  LowerLimitTransitionRegionWidth=0.1  LowerLimitTransitionRegionWidthUnits=deg  UpperLimitSpecify=off  UpperLimitBound=90  UpperLimitBoundUnits=deg  UpperLimitStiffness=1e4  UpperLimitStiffnessUnits=N*m/deg  UpperLimitDamping=10  UpperLimitDampingUnits=N*m/(deg/s)  UpperLimitTransitionRegionWidth=0.1  UpperLimitTransitionRegionWidthUnits=deg  TorqueActuationMode=ComputedTorque  MotionActuationMode=InputMotion  SensePosition=off  SenseVelocity=off  SenseAcceleration=off  SenseTorqueForce=off  SenseLowerLimitTorqueForce=off  SenseUpperLimitTorqueForce=off
  MechanismConfiguration : sm_lib/Utilities/Mechanism Configuration  UniformGravity=Constant  GravityVector=[0 0 -9.80665]  GravityVectorUnits=m/s^2  LinearizationDelta=0.001  JointModeTransitionNonlinearIterations=2
  Origin : sm_lib/Frames and Transforms/World Frame
  PS-Simulink Converter : nesl_utility/PS-Simulink Converter  PhysicalDomain=network_engine_domain  SubClassName=ps_output  LeftPortType=input  RightPortType=output  PseudoPeriodic=off  Frequencies=[]  VectorFormat=inherit  Unit=deg  AffineConversion=off
  Right Motor : sm_lib/Body Elements/File Solid  ExtGeomFileName=motor_Default_sldprt.STEP  UnitType=FromFile  ExtGeomFileUnits=m  StepReaderType=HEX  ExportConvexHullGeometry=off  InertiaType=CalculateFromGeometry  BasedOnType=Mass  Density=1000  DensityUnits=kg/m^3  Mass=MassVals.Motor  MassUnits=g  CenterOfMass=smiData.Solid(20).CoM  CenterOfMassUnits=mm  MomentsOfInertia=smiData.Solid(20).MoI  MomentsOfInertiaUnits=kg*mm^2  ProductsOfInertia=smiData.Solid(20).PoI  ProductsOfInertiaUnits=kg*mm^2  GraphicType=FromGeometry  MarkerShape=Sphere  MarkerSize=10  GraphicVisPropType=SimpleVisualProperties  GraphicDiffuseColor=[0.502 0.502 0.502]  GraphicOpacity=1  GraphicSpecularColor=[0.5 0.5 0.5 1.0]  GraphicAmbientColor=[0.15 0.15 0.15 1.0]  GraphicEmissiveColor=[0.0 0.0 0.0 1.0]  GraphicShininess=75  DoExposeReferenceFrame=off  SerializedFrames=|
      | <Frames>
      | 
      |   <Frame>
      |     <Id>Frame1</Id>
      |     <Value>
      |       <Name>Top</Name>
      |       <Origin>
      |         <Source>GeometricFeature</Source>
      |         <FeatureName>planar surface 1</FeatureName>
      |       </Origin>
      |       <PrimaryAxis>
      |         <DefinedDirection>+Y</DefinedDirection>
      |         <Source>ReferenceFrame</Source>
      |         <SourceDirection>+Z</SourceDirection>
      |         <FeatureName></FeatureName>
      |       </PrimaryAxis>
      |       <SecondaryAxis>
      |         <DefinedDirection>+X</DefinedDirection>
      |         <Source>ReferenceFrame</Source>
      |         <SourceDirection>-X</SourceDirection>
      |         <FeatureName></FeatureName>
      |       </SecondaryAxis>
      |     </Value>
      |   </Frame>
      | 
      | </Frames>
  Right Prop : sm_lib/Body Elements/File Solid  ExtGeomFileName=PropellerRED_Default_sldprt.STEP  UnitType=FromFile  ExtGeomFileUnits=m  StepReaderType=HEX  ExportConvexHullGeometry=off  InertiaType=CalculateFromGeometry  BasedOnType=Mass  Density=1000  DensityUnits=kg/m^3  Mass=MassVals.Prop  MassUnits=g  CenterOfMass=smiData.Solid(2).CoM  CenterOfMassUnits=mm  MomentsOfInertia=smiData.Solid(2).MoI  MomentsOfInertiaUnits=kg*mm^2  ProductsOfInertia=smiData.Solid(2).PoI  ProductsOfInertiaUnits=kg*mm^2  GraphicType=FromGeometry  MarkerShape=Sphere  MarkerSize=10  GraphicVisPropType=SimpleVisualProperties  GraphicDiffuseColor=[1 0 0]  GraphicOpacity=1  GraphicSpecularColor=[0.5 0.5 0.5 1.0]  GraphicAmbientColor=[0.15 0.15 0.15 1.0]  GraphicEmissiveColor=[0.0 0.0 0.0 1.0]  GraphicShininess=75  DoExposeReferenceFrame=off  SerializedFrames=|
      | <Frames>
      | 
      |   <Frame>
      |     <Id>Frame1</Id>
      |     <Value>
      |       <Name>Base</Name>
      |       <Origin>
      |         <Source>GeometricFeature</Source>
      |         <FeatureName>planar surface 3</FeatureName>
      |       </Origin>
      |       <PrimaryAxis>
      |         <DefinedDirection>+Z</DefinedDirection>
      |         <Source>ReferenceFrame</Source>
      |         <SourceDirection>+Z</SourceDirection>
      |         <FeatureName></FeatureName>
      |       </PrimaryAxis>
      |       <SecondaryAxis>
      |         <DefinedDirection>+X</DefinedDirection>
      |         <Source>ReferenceFrame</Source>
      |         <SourceDirection>+X</SourceDirection>
      |         <FeatureName></FeatureName>
      |       </SecondaryAxis>
      |     </Value>
      |   </Frame>
      | 
      | </Frames>
  Right Prop Axel : sm_lib/Joints/Revolute Joint  JointMode=Normal  CompositeWrenchDir=FollowerOnBase  CompositeWrenchFrame=BaseFrame  SenseConstraintForce=off  SenseConstraintTorque=off  SenseTotalForce=off  SenseTotalTorque=off  PositionTargetSpecify=on  PositionTargetPriority=Low  PositionTargetValue=0  PositionTargetValueUnits=deg  VelocityTargetSpecify=off  VelocityTargetPriority=High  VelocityTargetValue=0  VelocityTargetValueUnits=deg/s  EquilibriumPosition=0  EquilibriumPositionUnits=deg  SpringStiffness=0  SpringStiffnessUnits=N*m/deg  DampingCoefficient=0  DampingCoefficientUnits=N*m/(deg/s)  LowerLimitSpecify=off  LowerLimitBound=-90  LowerLimitBoundUnits=deg  LowerLimitStiffness=1e4  LowerLimitStiffnessUnits=N*m/deg  LowerLimitDamping=10  LowerLimitDampingUnits=N*m/(deg/s)  LowerLimitTransitionRegionWidth=0.1  LowerLimitTransitionRegionWidthUnits=deg  UpperLimitSpecify=off  UpperLimitBound=90  UpperLimitBoundUnits=deg  UpperLimitStiffness=1e4  UpperLimitStiffnessUnits=N*m/deg  UpperLimitDamping=10  UpperLimitDampingUnits=N*m/(deg/s)  UpperLimitTransitionRegionWidth=0.1  UpperLimitTransitionRegionWidthUnits=deg  TorqueActuationMode=ComputedTorque  MotionActuationMode=InputMotion  SensePosition=off  SenseVelocity=off  SenseAcceleration=off  SenseTorqueForce=off  SenseLowerLimitTorqueForce=off  SenseUpperLimitTorqueForce=off
  Rigid Transform : sm_lib/Frames and Transforms/Rigid Transform  RotationMethod=StandardAxis  FollAlignAxisA=+X  BaseAlignAxisA=+Y  FollAlignAxisB=+Y  BaseAlignAxisB=+Z  RotationStandardAxis=+X  RotationAngle=90  RotationAngleUnits=deg  RotationArbitraryAxis=[0 0 1]  RotationSequenceAxes=FollowerAxes  RotationSequence=XYX  RotationSequenceAngles=[0 0 0]  RotationSequenceAnglesUnits=deg  RotationMatrix=[1 0 0;0 1 0;0 0 1]  Quaternion=[1 0 0 0]  TranslationMethod=None  TranslationCartesianOffset=[0 0 0]  TranslationCartesianOffsetUnits=m  TranslationStandardAxis=+Z  TranslationStandardOffset=0  TranslationStandardOffsetUnits=m  TranslationROffset=0  TranslationROffsetUnits=m  TranslationThetaOffset=0  TranslationThetaOffsetUnits=deg  TranslationZOffset=0  TranslationZOffsetUnits=m
  Rigid Transform1 : sm_lib/Frames and Transforms/Rigid Transform  RotationMethod=StandardAxis  FollAlignAxisA=+X  BaseAlignAxisA=+Y  FollAlignAxisB=+Y  BaseAlignAxisB=+Z  RotationStandardAxis=+X  RotationAngle=90  RotationAngleUnits=deg  RotationArbitraryAxis=[0 0 1]  RotationSequenceAxes=FollowerAxes  RotationSequence=XYX  RotationSequenceAngles=[0 0 0]  RotationSequenceAnglesUnits=deg  RotationMatrix=[1 0 0;0 1 0;0 0 1]  Quaternion=[1 0 0 0]  TranslationMethod=None  TranslationCartesianOffset=[0 0 0]  TranslationCartesianOffsetUnits=m  TranslationStandardAxis=+Z  TranslationStandardOffset=0  TranslationStandardOffsetUnits=m  TranslationROffset=0  TranslationROffsetUnits=m  TranslationThetaOffset=0  TranslationThetaOffsetUnits=deg  TranslationZOffset=0  TranslationZOffsetUnits=m
  Rigid Transform2 : sm_lib/Frames and Transforms/Rigid Transform  RotationMethod=StandardAxis  FollAlignAxisA=+X  BaseAlignAxisA=+Y  FollAlignAxisB=+Y  BaseAlignAxisB=+Z  RotationStandardAxis=-X  RotationAngle=90  RotationAngleUnits=deg  RotationArbitraryAxis=[0 0 1]  RotationSequenceAxes=FollowerAxes  RotationSequence=XYX  RotationSequenceAngles=[0 0 0]  RotationSequenceAnglesUnits=deg  RotationMatrix=[1 0 0;0 1 0;0 0 1]  Quaternion=[1 0 0 0]  TranslationMethod=None  TranslationCartesianOffset=[0 0 0]  TranslationCartesianOffsetUnits=m  TranslationStandardAxis=+Z  TranslationStandardOffset=0  TranslationStandardOffsetUnits=m  TranslationROffset=0  TranslationROffsetUnits=m  TranslationThetaOffset=0  TranslationThetaOffsetUnits=deg  TranslationZOffset=0  TranslationZOffsetUnits=m
  Rigid Transform3 : sm_lib/Frames and Transforms/Rigid Transform  RotationMethod=StandardAxis  FollAlignAxisA=+X  BaseAlignAxisA=+Y  FollAlignAxisB=+Y  BaseAlignAxisB=+Z  RotationStandardAxis=-X  RotationAngle=90  RotationAngleUnits=deg  RotationArbitraryAxis=[0 0 1]  RotationSequenceAxes=FollowerAxes  RotationSequence=XYX  RotationSequenceAngles=[0 0 0]  RotationSequenceAnglesUnits=deg  RotationMatrix=[1 0 0;0 1 0;0 0 1]  Quaternion=[1 0 0 0]  TranslationMethod=None  TranslationCartesianOffset=[0 0 0]  TranslationCartesianOffsetUnits=m  TranslationStandardAxis=+Z  TranslationStandardOffset=0  TranslationStandardOffsetUnits=m  TranslationROffset=0  TranslationROffsetUnits=m  TranslationThetaOffset=0  TranslationThetaOffsetUnits=deg  TranslationZOffset=0  TranslationZOffsetUnits=m
  Stand : sm_lib/Body Elements/File Solid  ExtGeomFileName=stand_Default_sldprt.STEP  UnitType=FromFile  ExtGeomFileUnits=m  StepReaderType=HEX  ExportConvexHullGeometry=off  InertiaType=CalculateFromGeometry  BasedOnType=Mass  Density=1000  DensityUnits=kg/m^3  Mass=MassVals.Stand  MassUnits=g  CenterOfMass=smiData.Solid(21).CoM  CenterOfMassUnits=mm  MomentsOfInertia=smiData.Solid(21).MoI  MomentsOfInertiaUnits=kg*mm^2  ProductsOfInertia=smiData.Solid(21).PoI  ProductsOfInertiaUnits=kg*mm^2  GraphicType=FromGeometry  MarkerShape=Sphere  MarkerSize=10  GraphicVisPropType=SimpleVisualProperties  GraphicDiffuseColor=[0.3373 0.3373 0.3373]  GraphicOpacity=1  GraphicSpecularColor=[0.5 0.5 0.5 1.0]  GraphicAmbientColor=[0.15 0.15 0.15 1.0]  GraphicEmissiveColor=[0.0 0.0 0.0 1.0]  GraphicShininess=75  DoExposeReferenceFrame=off  SerializedFrames=|
      | <Frames>
      | 
      |   <Frame>
      |     <Id>Frame1</Id>
      |     <Value>
      |       <Name>Pivot</Name>
      |       <Origin>
      |         <Source>GeometricFeature</Source>
      |         <FeatureName>circular curve 8</FeatureName>
      |       </Origin>
      |       <PrimaryAxis>
      |         <DefinedDirection>+Z</DefinedDirection>
      |         <Source>ReferenceFrame</Source>
      |         <SourceDirection>+Z</SourceDirection>
      |         <FeatureName></FeatureName>
      |       </PrimaryAxis>
      |       <SecondaryAxis>
      |         <DefinedDirection>+X</DefinedDirection>
      |         <Source>ReferenceFrame</Source>
      |         <SourceDirection>+X</SourceDirection>
      |         <FeatureName></FeatureName>
      |       </SecondaryAxis>
      |     </Value>
      |   </Frame>
      | 
      |   <Frame>
      |     <Id>Frame2</Id>
      |     <Value>
      |       <Name>Base</Name>
      |       <Origin>
      |         <Source>GeometricFeature</Source>
      |         <FeatureName>planar surface 15</FeatureName>
      |       </Origin>
      |       <PrimaryAxis>
      |         <DefinedDirection>+Y</DefinedDirection>
      |         <Source>ReferenceFrame</Source>
      |         <SourceDirection>-Z</SourceDirection>
      |         <FeatureName></FeatureName>
      |       </PrimaryAxis>
      |       <SecondaryAxis>
      |         <DefinedDirection>+X</DefinedDirection>
      |         <Source>ReferenceFrame</Source>
      |         <SourceDirection>+X</SourceDirection>
      |         <FeatureName></FeatureName>
      |       </SecondaryAxis>
      |     </Value>
      |   </Frame>
      | 
      | </Frames>
  Stand-Body Pivot : sm_lib/Joints/Revolute Joint  JointMode=Normal  CompositeWrenchDir=FollowerOnBase  CompositeWrenchFrame=BaseFrame  SenseConstraintForce=off  SenseConstraintTorque=off  SenseTotalForce=off  SenseTotalTorque=off  PositionTargetSpecify=on  PositionTargetPriority=Low  PositionTargetValue=initial_angle  PositionTargetValueUnits=deg  VelocityTargetSpecify=off  VelocityTargetPriority=High  VelocityTargetValue=0  VelocityTargetValueUnits=deg/s  EquilibriumPosition=0  EquilibriumPositionUnits=deg  SpringStiffness=0  SpringStiffnessUnits=N*m/deg  DampingCoefficient=TwinPivotDamping  DampingCoefficientUnits=N*m/(deg/s)  LowerLimitSpecify=on  LowerLimitBound=-45  LowerLimitBoundUnits=deg  LowerLimitStiffness=1e3  LowerLimitStiffnessUnits=N*m/deg  LowerLimitDamping=1  LowerLimitDampingUnits=N*m/(deg/s)  LowerLimitTransitionRegionWidth=10  LowerLimitTransitionRegionWidthUnits=deg  UpperLimitSpecify=on  UpperLimitBound=45  UpperLimitBoundUnits=deg  UpperLimitStiffness=1e3  UpperLimitStiffnessUnits=N*m/deg  UpperLimitDamping=1  UpperLimitDampingUnits=N*m/(deg/s)  UpperLimitTransitionRegionWidth=10  UpperLimitTransitionRegionWidthUnits=deg  TorqueActuationMode=InputTorque  MotionActuationMode=ComputedMotion  SensePosition=on  SenseVelocity=off  SenseAcceleration=off  SenseTorqueForce=off  SenseLowerLimitTorqueForce=off  SenseUpperLimitTorqueForce=off
  Left Prop Position : PMIOPort  Side=Left
  Torque : PMIOPort  Port=2  Side=Left
  Right Prop Position : PMIOPort  Port=3  Side=Left
  Copter Angle : Outport
  wires:
  PS-Simulink Converter/1 -> Copter Angle/1
  connections:
  Origin/RConn1 -- Stand/RConn1 -- MechanismConfiguration/RConn1
  Stand/LConn1 -- Stand-Body Pivot/LConn1
  Body/LConn2 -- Stand-Body Pivot/RConn1
  Stand-Body Pivot/LConn2 -- Torque/RConn1
  Stand-Body Pivot/RConn2 -- PS-Simulink Converter/LConn1
  Right Prop Axel/LConn2 -- Right Prop Position/RConn1
  Left Prop Axel/LConn2 -- Left Prop Position/RConn1
  Rigid Transform/RConn1 -- Left Prop Axel/LConn1
  Left Prop/LConn1 -- Rigid Transform2/RConn1
  Right Prop/LConn1 -- Rigid Transform1/LConn1
  Left Prop Axel/RConn1 -- Rigid Transform2/LConn1
  Body/RConn1 -- Left Motor/LConn1 -- Rigid Transform/LConn1
  Rigid Transform1/RConn1 -- Right Prop Axel/RConn1
  Rigid Transform3/LConn1 -- Right Prop Axel/LConn1
  Rigid Transform3/RConn1 -- Body/LConn1 -- Right Motor/LConn1
